simulink model "lo_osc_normal_counter_test"  (Simulink 7.2)
settings: Solver=VariableStepDiscrete  StartTime=0.0  StopTime=1000  RelTol=1e-3
libraries: xbsIndex_r4 x7
settings Model: Creator=User  LastModifiedBy=root
settings OptimizationCC: InitFltsAndDblsToZero=on
settings DebuggingCC: SaveWithDisabledLinksMsg=none  SaveWithParameterizedLinksMsg=none

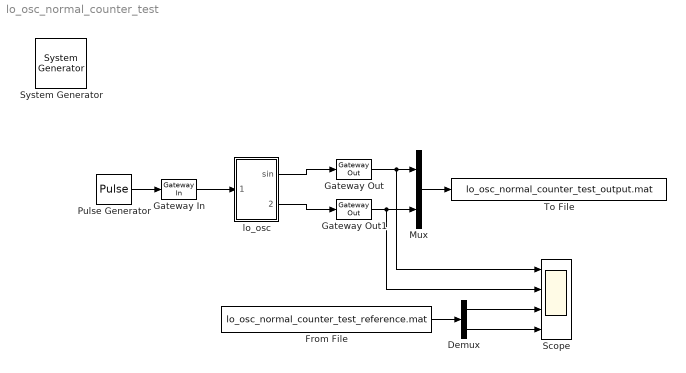
== system lo_osc_normal_counter_test ==
  " System Generator" : xbsIndex_r4/ System Generator  Tag=genX  SystemSampleTime=-1  xilinxfamily=Virtex4  part=xc4vsx35  speed=-10  package=ff668  synthesis_tool=XST  clock_wrapper=Clock Enables  directory=./netlist  testbench=off  simulink_period=1  sysclk_period=100  dcm_input_clock_period=100  incr_netlist=off  trim_vbits=Everywhere in SubSystem  dbl_ovrd=According to Block Masks  core_generation=According to Block Masks  run_coregen=off  deprecated_control=off  eval_field=0  block_type=sysgen
      settings: block_version=10.1.1
  Demux : Demux  Outputs=2
  From File : FromFile  FileName=lo_osc_normal_counter_test_reference.mat  SampleTime=1
  Gateway In : xbsIndex_r4/Gateway In  arith_type=Boolean  n_bits=16  bin_pt=14  quantization="Round  (unbiased: +/- Inf)"  overflow=Saturate  period=1  dbl_ovrd=off  timing_constraint=None  locs_specified=off  LOCs={}  hdl_port=on  block_type=gatewayin
      settings: infoedit="Gateway in block.  Converts inputs of type Simulink integer, double and fixed point to  Xilinx fixed point type.<br><br>Hardware notes:  In hardware these blocks become top level input ports."  block_version=11.4
  Gateway Out : xbsIndex_r4/Gateway Out  hdl_port=on  timing_constraint=None  locs_specified=off  LOCs={}  block_type=gatewayout
      settings: infoedit="Gateway out block.  Converts Xilinx fixed point inputs into ouputs of type Simulink integer, double, or fixed point.<P><P>Hardware notes:  In hardware these blocks become top level output ports or are discarded, depending on how they are configured."  block_version=10.1.1
  Gateway Out1 : xbsIndex_r4/Gateway Out  hdl_port=on  timing_constraint=None  locs_specified=off  LOCs={}  block_type=gatewayout
      settings: infoedit="Gateway out block.  Converts Xilinx fixed point inputs into ouputs of type Simulink integer, double, or fixed point.<P><P>Hardware notes:  In hardware these blocks become top level output ports or are discarded, depending on how they are configured."  block_version=10.1.1
  Mux : Mux  Inputs=2
  Pulse Generator : DiscretePulseGenerator  Period=100
  Scope : Scope  NumInputPorts=4
      settings: YMin=-5~-5~-5~-5  YMax=5~5~5~5
  To File : ToFile  Filename=lo_osc_normal_counter_test_output.mat  MatrixName=output
  lo_osc : Subsystem  mask(lo_osc){n_bits=10, counter_step=4, counter_start=3, counter_width=8, latency=3}
      mask prompts: n_bits "Output Bitwidth"; counter_step "counter step"; counter_start "counter start value"; counter_width "Counter Bitwidth"; latency "Lookup latency"
      mask help:
      | Generates -sin and cos data using a look-up
      | table.
      mask init:
      | lo_osc_init(gcb, ...
      |     'n_bits', n_bits, ...
      |     'counter_step', counter_step, ...
      |     'counter_start', counter_start, ...
      |     'counter_width', counter_width, ...
      |     'latency', latency);
      mask Help: eval('xlWeb(''http://casper.berkeley.edu/wiki/Lo_osc'')')
  wires:
  Gateway Out/1 -> Mux/1, Scope/1
  Gateway Out1/1 -> Mux/2, Scope/2
  lo_osc/1(sin) -> Gateway Out/1
  lo_osc/2(cos) -> Gateway Out1/1
  Mux/1 -> To File/1
  From File/1 -> Demux/1
  Demux/1 -> Scope/3
  Demux/2 -> Scope/4
  Pulse Generator/1 -> Gateway In/1
  Gateway In/1 -> lo_osc/1(sync)

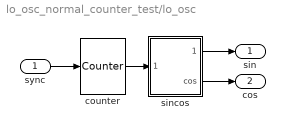
== system lo_osc_normal_counter_test/lo_osc ==
  sync : Inport  OutDataType=sfix(16)  OutScaling=2^0
  counter : xbsIndex_r4/Counter  cnt_type=Free Running  cnt_to=Inf  operation=Up  start_count=counter_start  cnt_by_val=counter_step  arith_type=Unsigned  n_bits=counter_width  bin_pt=0  load_pin=off  rst=on  en=off  explicit_period=on  period=1  dbl_ovrd=off  use_behavioral_HDL=off  implementation=Fabric  use_rpm=off  block_type=counter
  sincos : Subsystem  AncestorBlock=casper_library_downconverter/sincos  mask(sincos){func=sine and cosine, neg_sin=on, neg_cos=off, symmetric=off, handle_sync=off, depth_bits=8, bit_width=10, bram_latency=3}
      mask prompts: func "Function"; neg_sin "Negative sine"; neg_cos "Negative cosine"; symmetric "Symmetric output"; handle_sync "Handle sync"; depth_bits "Lookup table depth (2^?)"; bit_width "Output bit width"; bram_latency "BRAM latency"
      mask init:
      | sincos_init(gcb, ...
      |     'func', func, ...
      |     'neg_sin', neg_sin, ...
      |     'neg_cos', neg_cos, ...
      |     'symmetric', symmetric, ...
      |     'handle_sync', handle_sync, ...
      |     'depth_bits', depth_bits, ...
      |     'bit_width', bit_width, ...
      |     'bram_latency', bram_latency);
      mask StyleString: popup(cosine|sine|sine and cosine),checkbox,checkbox,checkbox,checkbox,edit,edit,edit
  sin : Outport  OutDataType=sfix(16)  OutScaling=2^0
  cos : Outport  Port=2  OutDataType=sfix(16)  OutScaling=2^0
  wires:
  sincos/1(-sine) -> sin/1
  sincos/2(cos) -> cos/1
  counter/1 -> sincos/1(theta)
  sync/1 -> counter/1

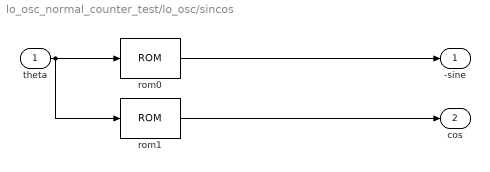
== system lo_osc_normal_counter_test/lo_osc/sincos ==
  theta : Inport
  rom0 : xbsIndex_r4/ROM  depth=2^depth_bits  initVector=-sin(2*pi*(0:(2^depth_bits-1))/(2^depth_bits))  distributed_mem=Block RAM  rst=off  init_reg=0  en=off  latency=bram_latency  arith_type="Signed  (2's comp)"  n_bits=bit_width  bin_pt=bit_width-1  dbl_ovrd=off  optimize=Area  use_rpm=on  block_type=sprom
      settings: block_version=10.1.3
  rom1 : xbsIndex_r4/ROM  depth=2^depth_bits  initVector=cos(2*pi*(0:(2^depth_bits-1))/(2^depth_bits))  distributed_mem=Block RAM  rst=off  init_reg=0  en=off  latency=bram_latency  arith_type="Signed  (2's comp)"  n_bits=bit_width  bin_pt=bit_width-1  dbl_ovrd=off  optimize=Area  use_rpm=on  block_type=sprom
      settings: block_version=10.1.3
  -sine : Outport
  cos : Outport  Port=2
  wires:
  theta/1 -> rom0/1, rom1/1
  rom0/1 -> -sine/1
  rom1/1 -> cos/1
